simulink model "quadrotor_model"  (R2024b)
settings: Solver=VariableStepAuto  StartTime=0.0  StopTime=15  FixedStep=0.005  RelTol=1e-3
values from neighbouring files (symbols this model uses):
  Kd_phi = Cphi.Kd    [pidtune_baseline.m]
  Kd_psi = Cpsi.Kd    [pidtune_baseline.m]
  Kd_theta = Ctheta.Kd    [pidtune_baseline.m]
  Kd_z = Cz.Kd    [pidtune_baseline.m]
  Ki_phi = Cphi.Ki    [pidtune_baseline.m]
  Ki_psi = Cpsi.Ki    [pidtune_baseline.m]
  Ki_theta = Ctheta.Ki    [pidtune_baseline.m]
  Ki_z = Cz.Ki    [pidtune_baseline.m]
  Kp_phi = Cphi.Kp    [pidtune_baseline.m]
  Kp_psi = Cpsi.Kp    [pidtune_baseline.m]
  Kp_theta = Ctheta.Kp    [pidtune_baseline.m]
  Kp_z = Cz.Kp    [pidtune_baseline.m]
  l = 0.225    [motor_forward.m]
undefined symbols (not defined in the file or in its folder): altitude_d, altitude_i, b, g, I_xx, I_yy, I_zz, Im, k, m, pitch_d, pitch_i, roll_d, roll_i, yaw_d, yaw_i
libraries: slpidlib x4
settings Model: Creator=angel  LastModifiedBy=Yusuf
settings SolverCC: AlgebraicLoopSolver=TrustRegion
settings DataIOCC: ReturnWorkspaceOutputs=off
settings DebuggingCC: UnconnectedInputMsg=warning  UnconnectedOutputMsg=warning  UnconnectedLineMsg=warning  ArithmeticOperatorsInVariantConditions=warning
settings ModelReferenceCC: EnableRefExpFcnMdlSchedulingChecks=on
settings SFSimCC: SimUseLocalCustomCode=off  CustomCodeUndefinedFunction=UseInterfaceOnly
settings RTWCC: RTWUseLocalCustomCode=off  GPUComputeCapability=3.5
settings CodeAppCC: StateflowObjectComments=on

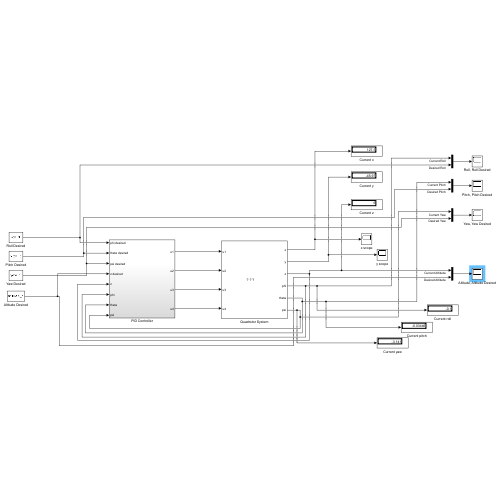
[thumbnail: Simulink's stored preview of the top-level diagram]
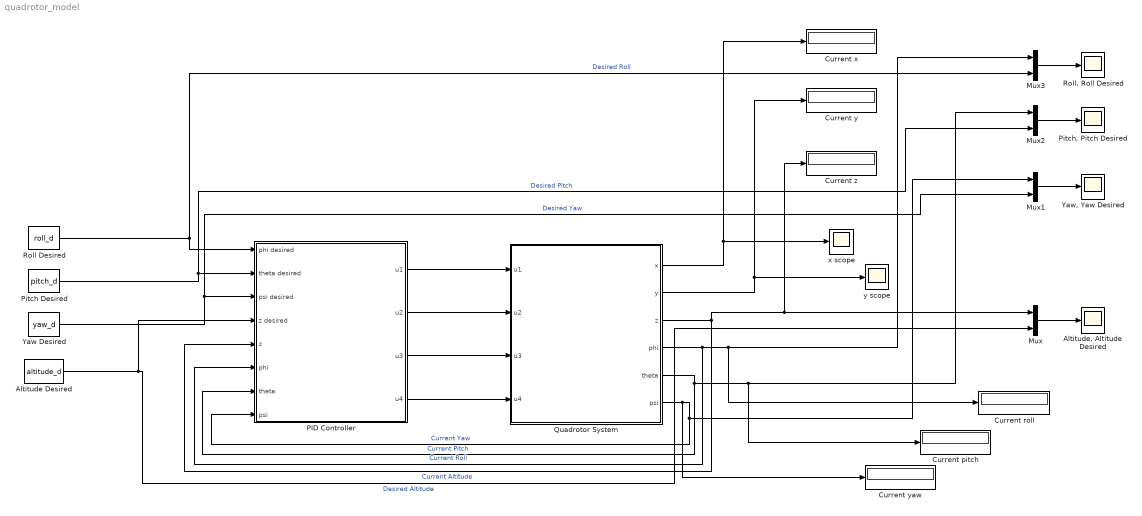
== system quadrotor_model ==
  Altitude Desired : Constant  Value=altitude_d
  "Altitude, Altitude Desired" : Scope
  Current pitch : Display
  Current roll : Display
  Current x : Display
  Current y : Display
  Current yaw : Display
  Current z : Display
  Mux{,1..3} (4 alike) : Mux  Inputs=2
  PID Controller : Subsystem
  Pitch Desired : Constant  Value=pitch_d
  "Pitch, Pitch Desired" : Scope
  Quadrotor System : Subsystem
      mask Display: image('C:\Users\angel\OneDrive - Universidad Politécnica de Yucatán\CIMAT\1st semester\Robotic Systems Modeling and Control\Project\Quadrotor\images\quadrotor.jpg');
  Roll Desired : Constant  Value=roll_d
  "Roll, Roll Desired" : Scope
  Yaw Desired : Constant  Value=yaw_d
  "Yaw, Yaw Desired" : Scope
  x scope : Scope
  y scope : Scope
  wires:
  Quadrotor System/1(x) -> x scope/1, Current x/1
  Quadrotor System/2(y) -> Current y/1, y scope/1
  Quadrotor System/3(z) -> Current z/1, Mux/1, PID Controller/5(z)  "Current Altitude"
  Quadrotor System/5(theta) -> Mux2/1, Current pitch/1, PID Controller/7(theta)  "Current Pitch"
  Quadrotor System/6(psi) -> Current yaw/1, Mux1/1, PID Controller/8(psi)  "Current Yaw"
  Mux/1 -> "Altitude, Altitude Desired"/1
  Roll Desired/1 -> Mux3/2, PID Controller/1(phi desired)  "Desired Roll"
  Pitch Desired/1 -> Mux2/2, PID Controller/2(theta desired)  "Desired Pitch"
  Yaw Desired/1 -> Mux1/2, PID Controller/3(psi desired)  "Desired Yaw"
  Quadrotor System/4(phi) -> PID Controller/6(phi), Current roll/1, Mux3/1  "Current Roll"
  Mux2/1 -> "Pitch, Pitch Desired"/1
  Mux1/1 -> "Yaw, Yaw Desired"/1
  Mux3/1 -> "Roll, Roll Desired"/1
  Altitude Desired/1 -> PID Controller/4(z desired), Mux/2  "Desired Altitude"
  PID Controller/1(u1) -> Quadrotor System/1(u1)
  PID Controller/2(u2) -> Quadrotor System/2(u2)
  PID Controller/3(u3) -> Quadrotor System/3(u3)
  PID Controller/4(u4) -> Quadrotor System/4(u4)

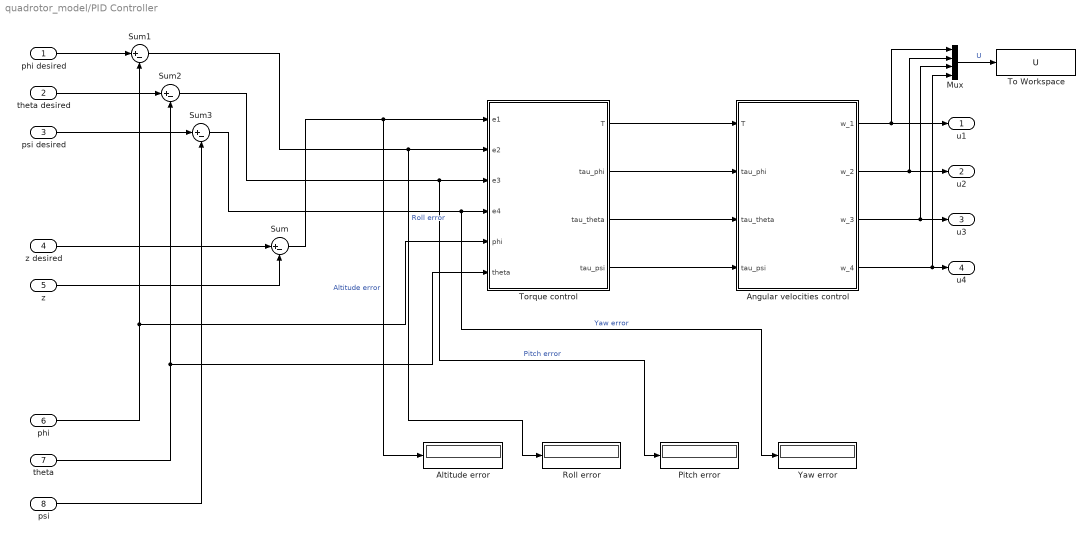
== system quadrotor_model/PID Controller ==
  phi desired : Inport
  theta desired : Inport  Port=2
  psi desired : Inport  Port=3
  z desired : Inport  Port=4
  z : Inport  Port=5
  phi : Inport  Port=6
  theta : Inport  Port=7
  psi : Inport  Port=8
  Altitude error : Display
  Angular velocities control : Subsystem
  Mux : Mux
  Pitch error : Display
  Roll error : Display
  Sum{,1..3} (4 alike) : Sum  Inputs=|+-
  To Workspace : ToWorkspace  VariableName=U  SaveFormat=Timeseries  SampleTime=-1
  Torque control : Subsystem
  Yaw error : Display
  u1 : Outport
  u2 : Outport  Port=2
  u3 : Outport  Port=3
  u4 : Outport  Port=4
  wires:
  z desired/1 -> Sum/1
  z/1 -> Sum/2
  Sum/1 -> Altitude error/1, Torque control/1(e1)  "Altitude error"
  phi desired/1 -> Sum1/1
  phi/1 -> Torque control/5("phi "), Sum1/2
  theta desired/1 -> Sum2/1
  theta/1 -> Sum2/2, Torque control/6("theta ")
  psi desired/1 -> Sum3/1
  psi/1 -> Sum3/2
  Sum1/1 -> Roll error/1, Torque control/2(e2)  "Roll error"
  Sum2/1 -> Pitch error/1, Torque control/3(e3)  "Pitch error"
  Sum3/1 -> Yaw error/1, Torque control/4(e4)  "Yaw error"
  Torque control/2(tau_phi) -> Angular velocities control/2(tau_phi)
  Torque control/1(T) -> Angular velocities control/1(T)
  Torque control/3(tau_theta) -> Angular velocities control/3(tau_theta)
  Torque control/4(tau_psi) -> Angular velocities control/4("tau_psi ")
  Angular velocities control/1(w_1) -> Mux/1, u1/1
  Angular velocities control/2(w_2) -> Mux/2, u2/1
  Angular velocities control/3(w_3) -> Mux/3, u3/1
  Angular velocities control/4("w_4 ") -> Mux/4, u4/1
  Mux/1 -> To Workspace/1  "U"

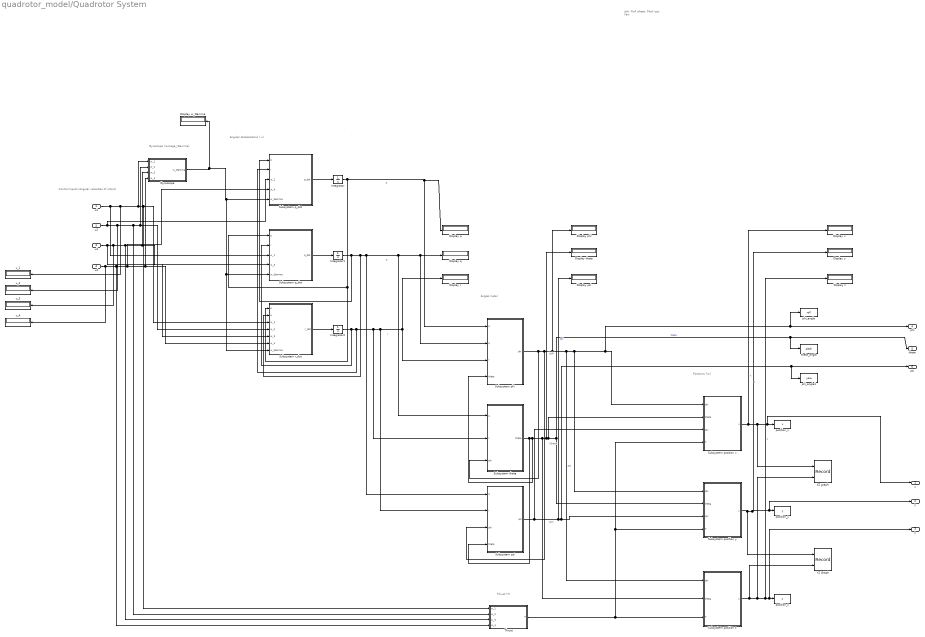
== system quadrotor_model/Quadrotor System ==
  note: Angular Accelerations (\nu)
  note: .
  note: \phi: Roll
      | \theta: Pitch
      | \psi: Yaw
  note: Control Inputs
      | (Angular velocities of rotors)
  note: Positions (\xi)
  note: Angles (\eta)
  note: Gyroscope (\omega_\Gamma)
  note: Thrust (T)
  note: p
  note: q
  note: r
  note: \phi
  note: \theta
  note: \psi
  u1 : Inport
  u2 : Inport  Port=2
  u3 : Inport  Port=3
  u4 : Inport  Port=4
  Display p : Display
  Display phi : Display
  Display psi : Display
  Display q : Display
  Display r : Display
  Display theta : Display
  Display w_Gamma : Display
  Display x : Display
  Display y : Display
  Display z : Display
  Gyroscope : MATLAB Function  TreatAsAtomicUnit=on
  Integrator : Integrator
  Integrator1 : Integrator
  Integrator2 : Integrator
  Subsystem p_dot : Subsystem
  Subsystem phi : Subsystem
  Subsystem position x : Subsystem
  Subsystem position y : Subsystem
  Subsystem position z : Subsystem
  Subsystem psi : Subsystem
  Subsystem q_dot : Subsystem
  Subsystem r_dot : Subsystem
  Subsystem theta : Subsystem
  Thrust : MATLAB Function  TreatAsAtomicUnit=on
  XZ graph : Record  FileSettingsInternal="{\"entries\":[{\"content\":{\"excelSettings\":{\"content\":{},\"type\":\"Streamout.ExcelSettings\"}},\"type\":\"Streamout.FileSettingStorage\",\"uuid\":\"\"}],\"packageUris\":[\"http:\\/\\/schema.mathworks.com\\/mf0\\/streamout_blocks\\/R2020a\"],\"version\":\"1.0\"}"  Layout=[1 1]  SignalsInternal="{\"entries\":[{\"content\":{\"signals\":[{\"content\":{\"blockPath\":[],\"dimensions\":[1],\"domain\":\"\",\"lineColor\":\"#a2142f\",\"plots\":[ 1 ],\"port\":1,\"sid\":[\"\"],\"signalID\":1,\"signalName\":\"x\"},\"type\":\"RecordBlkView.Signal\",\"uuid\":\"\"},{\"content\":{\"blockPath\":[],\"dimensions\":[1],\"domain\":\"\",\"lineColor\":\"#139fff\",\"plots\":[ 1 ],\"port\":2,\"sid\":[\"\"],\"signalID\":2,\"signalName\":\"z\"},\"type\":\"RecordBlkView.Signal\",\"uuid\":\"\"}]},\"type\":\"RecordBlkView.InputSignals\",\"uuid\":\"\"}],\"packageUris\":[\"http:\\/\\/schema.mathworks.com\\/mf0\\/streamout_blocks\\/R2020a\"],\"version\":\"1.0\"}"  VisualizationBindings="{\"xyplotplugin\":{\"info\":[{\"series\":[{\"bindingParametersList\":[{\"parameter\":\"X-Axis\",\"signalID\":1,\"signalName\":\"x\"},{\"parameter\":\"Y-Axis\",\"signalID\":2,\"signalName\":\"z\"}],\"seriesID\":0}],\"subplotID\":1}]}}"  CompatibilityTag=XY  st=-1
  YZ Graph : Record  FileSettingsInternal="{\"entries\":[{\"content\":{\"excelSettings\":{\"content\":{},\"type\":\"Streamout.ExcelSettings\"}},\"type\":\"Streamout.FileSettingStorage\",\"uuid\":\"\"}],\"packageUris\":[\"http:\\/\\/schema.mathworks.com\\/mf0\\/streamout_blocks\\/R2020a\"],\"version\":\"1.0\"}"  Layout=[1 1]  SignalsInternal="{\"entries\":[{\"content\":{\"signals\":[{\"content\":{\"blockPath\":[],\"dimensions\":[1],\"domain\":\"\",\"lineColor\":\"#a2142f\",\"plots\":[ 1 ],\"port\":1,\"sid\":[\"\"],\"signalID\":1,\"signalName\":\"y\"},\"type\":\"RecordBlkView.Signal\",\"uuid\":\"\"},{\"content\":{\"blockPath\":[],\"dimensions\":[1],\"domain\":\"\",\"lineColor\":\"#139fff\",\"plots\":[ 1 ],\"port\":2,\"sid\":[\"\"],\"signalID\":2,\"signalName\":\"z\"},\"type\":\"RecordBlkView.Signal\",\"uuid\":\"\"}]},\"type\":\"RecordBlkView.InputSignals\",\"uuid\":\"\"}],\"packageUris\":[\"http:\\/\\/schema.mathworks.com\\/mf0\\/streamout_blocks\\/R2020a\"],\"version\":\"1.0\"}"  VisualizationBindings="{\"xyplotplugin\":{\"info\":[{\"series\":[{\"bindingParametersList\":[{\"parameter\":\"X-Axis\",\"signalID\":1,\"signalName\":\"y\"},{\"parameter\":\"Y-Axis\",\"signalID\":2,\"signalName\":\"z\"}],\"seriesID\":0}],\"subplotID\":1}]}}"  CompatibilityTag=XY  st=-1
  phi_angle : ToWorkspace  VariableName=roll  SampleTime=-1
  phi_angle1 : ToWorkspace  VariableName=yaw  SampleTime=-1
  position_x : ToWorkspace  VariableName=x  SampleTime=-1
  position_y : ToWorkspace  VariableName=y  SampleTime=-1
  position_z : ToWorkspace  VariableName=z  SampleTime=-1
  theta_angle : ToWorkspace  VariableName=pitch  SampleTime=-1
  u_{1..4} (4 alike) : Display
  x : Outport
  y : Outport  Port=2
  z : Outport  Port=3
  phi : Outport  Port=4
  theta : Outport  Port=5
  psi : Outport  Port=6
  wires:
  u1/1 -> Subsystem q_dot/3(w_1), u_1/1, Gyroscope/1(w_1), Subsystem r_dot/3(w_1), Thrust/1(w_1)
  u2/1 -> Subsystem p_dot/3(w_2), u_2/1, Gyroscope/2(w_2), Subsystem r_dot/4(w_2), Thrust/2(w_2)
  u3/1 -> Subsystem q_dot/4(w_3), Gyroscope/3(w_3), Subsystem r_dot/5(w_3), Thrust/3(w_3), u_3/1
  u4/1 -> u_4/1, Gyroscope/4(w_4), Subsystem r_dot/6(w_4), Subsystem p_dot/4(w_4), Thrust/4(w_4)
  Thrust/1(T) -> Subsystem position y/4("T "), Subsystem position x/4(T), Subsystem position z/3(T)
  Subsystem phi/1("phi ") -> Subsystem theta/3("phi "), Subsystem psi/3(phi), Display phi/1, Subsystem position z/1("phi "), Subsystem position y/1("phi "), phi_angle/1, phi/1, Subsystem position x/1("phi ")  "phi"
  Subsystem psi/1(psi) -> Subsystem position x/3("psi "), Display psi/1, phi_angle1/1, psi/1, Subsystem position y/3("psi ")  "psi"
  Subsystem position x/1(x) -> Display x/1, x/1, position_x/1, XZ graph/1  "x"
  Subsystem position z/1(z) -> YZ Graph/2, XZ graph/2, z/1, position_z/1, Display z/1  "z"
  Subsystem position y/1("y ") -> y/1, position_y/1, Display y/1, YZ Graph/1  "y"
  Gyroscope/1(w_Gamma) -> Display w_Gamma/1, Subsystem r_dot/7(w_Gamma), Subsystem q_dot/5("w_Gamma "), Subsystem p_dot/5("w_Gamma ")
  Subsystem p_dot/1(p_dot) -> Integrator/1
  Subsystem q_dot/1(q_dot) -> Integrator1/1
  Subsystem r_dot/1(r_dot) -> Integrator2/1
  Integrator/1 -> Subsystem r_dot/1("p "), Subsystem q_dot/1("p "), Display p/1, Subsystem phi/1(p)
  Integrator2/1 -> Subsystem theta/2(r), Subsystem psi/2(r), Display r/1, Subsystem phi/3(r), Subsystem p_dot/2(r), Subsystem q_dot/2(r)
  Integrator1/1 -> Subsystem p_dot/1(q), Subsystem psi/1(q), Subsystem theta/1(q), Display q/1, Subsystem phi/2(q), Subsystem r_dot/2(q)
  Subsystem theta/1(theta) -> Subsystem psi/4(theta), Subsystem phi/4(theta), Subsystem position z/2("theta "), Display theta/1, Subsystem position x/2("theta "), theta_angle/1, theta/1, Subsystem position y/2("theta ")  "theta"

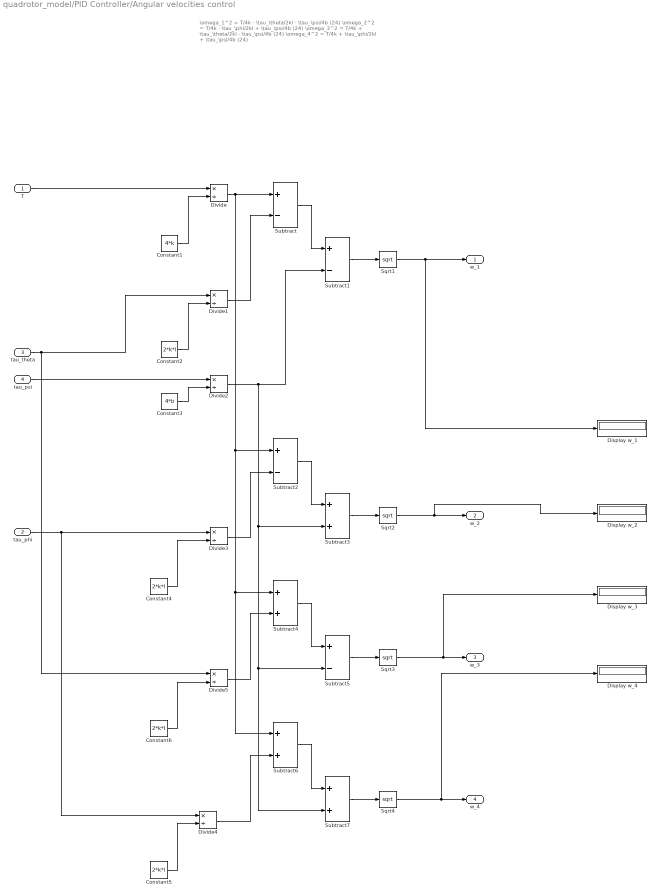
== system quadrotor_model/PID Controller/Angular velocities control ==
  note: \omega_1^2 = T/4k - \tau_\theta/2kl - \tau_\psi/4b   (24)
      |
      | \omega_2^2 = T/4k - \tau_\phi/2kl + \tau_\psi/4b   (24)
      |
      | \omega_3^2 = T/4k + \tau_\theta/2kl - \tau_\psi/4b   (24)
      |
      | \omega_4^2 = T/4k + \tau_\phi/2kl + \tau_\psi/4b   (24)
  T : Inport
  tau_phi : Inport  Port=2
  tau_theta : Inport  Port=3
  "tau_psi " : Inport  Port=4
  Constant1 : Constant  Value=4*k
  Constant{2,4..6} (4 alike) : Constant  Value=2*k*l
  Constant3 : Constant  Value=4*b
  Display w_{1..4} (4 alike) : Display
  Divide{,1..5} (6 alike) : Product  Inputs=*/
  Sqrt1 : Sqrt
  Sqrt2 : Sqrt  OutputSignalType=real
  Sqrt3 : Sqrt
  Sqrt4 : Sqrt
  Subtract{,1..2,5} (4 alike) : Sum  Inputs=+-
  Subtract{3..4,6..7} (4 alike) : Sum
  w_1 : Outport
  w_2 : Outport  Port=2
  w_3 : Outport  Port=3
  "w_4 " : Outport  Port=4
  wires:
  Constant1/1 -> Divide/2
  T/1 -> Divide/1
  Divide/1 -> Subtract4/1, Subtract6/1, Subtract2/1, Subtract/1
  Constant2/1 -> Divide1/2
  tau_theta/1 -> Divide5/1, Divide1/1
  Divide1/1 -> Subtract/2
  Subtract/1 -> Subtract1/1
  Constant3/1 -> Divide2/2
  Subtract1/1 -> Sqrt1/1
  Sqrt1/1 -> Display w_1/1, w_1/1
  Constant4/1 -> Divide3/2
  tau_phi/1 -> Divide4/1, Divide3/1
  Divide3/1 -> Subtract2/2
  Subtract2/1 -> Subtract3/1
  "tau_psi "/1 -> Divide2/1
  Divide2/1 -> Subtract7/2, Subtract5/2, Subtract3/2, Subtract1/2
  Sqrt2/1 -> Display w_2/1, w_2/1
  Subtract3/1 -> Sqrt2/1
  Constant6/1 -> Divide5/2
  Divide5/1 -> Subtract4/2
  Subtract5/1 -> Sqrt3/1
  Subtract4/1 -> Subtract5/1
  Sqrt3/1 -> Display w_3/1, w_3/1
  Subtract7/1 -> Sqrt4/1
  Constant5/1 -> Divide4/2
  Divide4/1 -> Subtract6/2
  Subtract6/1 -> Subtract7/1
  Sqrt4/1 -> Display w_4/1, "w_4 "/1

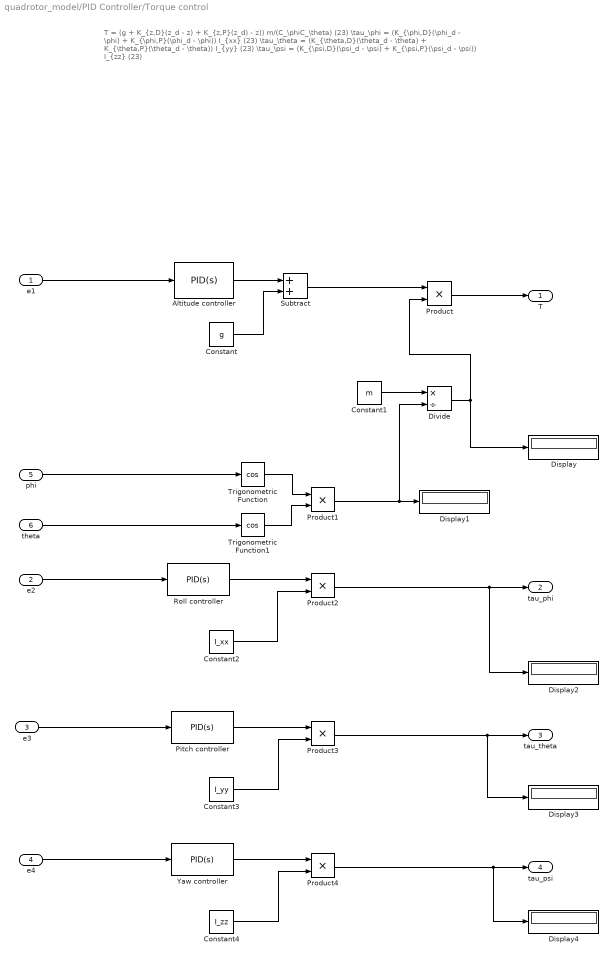
== system quadrotor_model/PID Controller/Torque control ==
  note: T = (g + K_{z,D}(z_d - z) + K_{z,P}(z_d) - z)) m/(C_\phiC_\theta)     (23)
      |
      | \tau_\phi = (K_{\phi,D}(\phi_d - \phi) + K_{\phi,P}(\phi_d - \phi)) I_{xx}                   (23)
      |
      | \tau_\theta = (K_{\theta,D}(\theta_d - \theta) + K_{\theta,P}(\theta_d - \theta)) I_{yy}                    (23)
      |
      | \tau_\psi = (K_{\psi,D}(\psi_d - \psi) + K_{\psi,P}(\psi_d - \psi)) I_{zz}                (23)
  e1 : Inport
  e2 : Inport  Port=2
  e3 : Inport  Port=3
  e4 : Inport  Port=4
  "phi " : Inport  Port=5
  "theta " : Inport  Port=6
  Altitude controller : slpidlib/PID Controller  Controller=PID  Form=Parallel  TimeDomain=Continuous-time  UseExternalTs=off  SampleTime=-1  IntegratorMethod=Forward Euler  FilterMethod=Forward Euler  ControllerParametersSource=internal  P=Kp_z  I=Ki_z  UseKiTs=off  D=Kd_z  UseExternalDerivativeSource=off  N=572.770791824146  UseFilter=on  TunerSelectOption=Transfer Function Based (PID Tuner App)  InitialConditionSource=internal  InitialConditionForIntegrator=0  InitialConditionForFilter=0  DifferentiatorICPrevScaledInput=0  ExternalReset=none  TrackingMode=off  Kt=1  LimitOutput=on  SatLimitsSource=internal  UpperSaturationLimit=5  LowerSaturationLimit=-5  LinearizeAsGain=on  AntiWindupMode=none  Kb=1  LimitIntegrator=off  UpperIntegratorSaturationLimit=inf  LowerIntegratorSaturationLimit=-inf  POutMin=[]  POutMax=[]  IOutMin=[]  IOutMax=[]  DOutMin=[]  DOutMax=[]  NOutMin=[]  NOutMax=[]  SumOutMin=[]  SumOutMax=[]  SaturationOutMin=[]  SaturationOutMax=[]  PParamMin=[]  PParamMax=[]  IParamMin=[]  IParamMax=[]  DParamMin=[]  DParamMax=[]  NParamMin=[]  NParamMax=[]  KbParamMin=[]  KbParamMax=[]  KtParamMin=[]  KtParamMax=[]  KbOutMin=[]  KbOutMax=[]  KtOutMin=[]  KtOutMax=[]  IntegratorOutMin=[]  IntegratorOutMax=[]  FilterOutMin=[]  FilterOutMax=[]  SumI1OutMin=[]  SumI1OutMax=[]  SumI2OutMin=[]  SumI2OutMax=[]  SumI3OutMin=[]  SumI3OutMax=[]  SumI4OutMin=[]  SumI4OutMax=[]  SumDOutMin=[]  SumDOutMax=[]  DifferentiatorOutMin=[]  DifferentiatorOutMax=[]  FilterDiffOutCoefMin=[]  FilterDiffOutCoefMax=[]  ReciprocalOutMin=[]  ReciprocalOutMax=[]  SumDenOutMin=[]  SumDenOutMax=[]  SumNumOutMin=[]  SumNumOutMax=[]  DivideOutMin=[]  DivideOutMax=[]  UdiffTsProdOutMin=[]  UdiffTsProdOutMax=[]  NTsProdOutMin=[]  NTsProdOutMax=[]  UintegralTsProdOutMin=[]  UintegralTsProdOutMax=[]  UngainTsProdOutMin=[]  UngainTsProdOutMax=[]  ClampingZeroOutDataTypeStr=Inherit: Inherit via back propagation  ClampingZeroOutMin=[]  ClampingZeroOutMax=[]  FilterDenConstantOutDataTypeStr=Inherit: Inherit via back propagation  FilterDenConstantOutMin=[]  FilterDenConstantOutMax=[]  PCopyOutDataTypeStr=Inherit: Inherit via back propagation  PCopyOutMin=[]  PCopyOutMax=[]  NCopyOutDataTypeStr=Inherit: Inherit via back propagation  NCopyOutMin=[]  NCopyOutMax=[]  IntegratorContinuousStateAttributes=''  IntegratorStateMustResolveToSignalObject=off  IntegratorRTWStateStorageClass=Auto  FilterContinuousStateAttributes=''  FilterStateMustResolveToSignalObject=off  FilterRTWStateStorageClass=Auto  ParallelPVariant=InternalParameters  IdealPVariant=Disabled  IVariant=InternalParameters  DVariant=InternalParameters  IntegratorVariant=Continuous  SatVariant=Enabled  AWVariant=Passthrough  PCopyVariant=Disabled  TRVariant=Disabled  FdbkBlocksVariant=Forward  IdealPFdbkVariant=Disabled  SatFdbkVariant=Disabled  DerivativeFilterVariant=ContFilter  NVariant=InternalParameters  NCopyVariant=Disabled  FilterICVariant=InternalICsFilter  IntegratorICVariant=InternalICs  ExternalResetVariant=Disabled  TRSumVariant=Passthrough  SumFdbkVariant=Disabled  SumVariant=Sum_PID  TsampFilterVariant=InternalTs  TsampNgainVariant=Passthrough  TsampIntegralVariant=Disabled_SignalSpec  ExternalSaturationOutDataTypeStr=Inherit: Same as second input  DerivativeSourceVariant=ErrorSignal  PreIntVariant=InternalPreInt
  Constant : Constant  Value=g
  Constant1 : Constant  Value=m
  Constant2 : Constant  Value=I_xx
  Constant3 : Constant  Value=I_yy
  Constant4 : Constant  Value=I_zz
  Display{,1..4} (5 alike) : Display
  Divide : Product  Inputs=*/
  Pitch controller : slpidlib/PID Controller  Controller=PID  Form=Parallel  TimeDomain=Continuous-time  UseExternalTs=off  SampleTime=-1  IntegratorMethod=Forward Euler  FilterMethod=Forward Euler  ControllerParametersSource=internal  P=Kp_theta  I=Ki_theta  UseKiTs=off  D=Kd_theta  UseExternalDerivativeSource=off  N=1414.64809761679  UseFilter=on  TunerSelectOption=Transfer Function Based (PID Tuner App)  InitialConditionSource=internal  InitialConditionForIntegrator=0  InitialConditionForFilter=0  DifferentiatorICPrevScaledInput=0  ExternalReset=none  TrackingMode=off  Kt=1  LimitOutput=on  SatLimitsSource=internal  UpperSaturationLimit=0.9  LowerSaturationLimit=-0.9  LinearizeAsGain=on  AntiWindupMode=none  Kb=1  LimitIntegrator=off  UpperIntegratorSaturationLimit=inf  LowerIntegratorSaturationLimit=-inf  POutMin=[]  POutMax=[]  IOutMin=[]  IOutMax=[]  DOutMin=[]  DOutMax=[]  NOutMin=[]  NOutMax=[]  SumOutMin=[]  SumOutMax=[]  SaturationOutMin=[]  SaturationOutMax=[]  PParamMin=[]  PParamMax=[]  IParamMin=[]  IParamMax=[]  DParamMin=[]  DParamMax=[]  NParamMin=[]  NParamMax=[]  KbParamMin=[]  KbParamMax=[]  KtParamMin=[]  KtParamMax=[]  KbOutMin=[]  KbOutMax=[]  KtOutMin=[]  KtOutMax=[]  IntegratorOutMin=[]  IntegratorOutMax=[]  FilterOutMin=[]  FilterOutMax=[]  SumI1OutMin=[]  SumI1OutMax=[]  SumI2OutMin=[]  SumI2OutMax=[]  SumI3OutMin=[]  SumI3OutMax=[]  SumI4OutMin=[]  SumI4OutMax=[]  SumDOutMin=[]  SumDOutMax=[]  DifferentiatorOutMin=[]  DifferentiatorOutMax=[]  FilterDiffOutCoefMin=[]  FilterDiffOutCoefMax=[]  ReciprocalOutMin=[]  ReciprocalOutMax=[]  SumDenOutMin=[]  SumDenOutMax=[]  SumNumOutMin=[]  SumNumOutMax=[]  DivideOutMin=[]  DivideOutMax=[]  UdiffTsProdOutMin=[]  UdiffTsProdOutMax=[]  NTsProdOutMin=[]  NTsProdOutMax=[]  UintegralTsProdOutMin=[]  UintegralTsProdOutMax=[]  UngainTsProdOutMin=[]  UngainTsProdOutMax=[]  ClampingZeroOutDataTypeStr=Inherit: Inherit via back propagation  ClampingZeroOutMin=[]  ClampingZeroOutMax=[]  FilterDenConstantOutDataTypeStr=Inherit: Inherit via back propagation  FilterDenConstantOutMin=[]  FilterDenConstantOutMax=[]  PCopyOutDataTypeStr=Inherit: Inherit via back propagation  PCopyOutMin=[]  PCopyOutMax=[]  NCopyOutDataTypeStr=Inherit: Inherit via back propagation  NCopyOutMin=[]  NCopyOutMax=[]  IntegratorContinuousStateAttributes=''  IntegratorStateMustResolveToSignalObject=off  IntegratorRTWStateStorageClass=Auto  FilterContinuousStateAttributes=''  FilterStateMustResolveToSignalObject=off  FilterRTWStateStorageClass=Auto  ParallelPVariant=InternalParameters  IdealPVariant=Disabled  IVariant=InternalParameters  DVariant=InternalParameters  IntegratorVariant=Continuous  SatVariant=Enabled  AWVariant=Passthrough  PCopyVariant=Disabled  TRVariant=Disabled  FdbkBlocksVariant=Forward  IdealPFdbkVariant=Disabled  SatFdbkVariant=Disabled  DerivativeFilterVariant=ContFilter  NVariant=InternalParameters  NCopyVariant=Disabled  FilterICVariant=InternalICsFilter  IntegratorICVariant=InternalICs  ExternalResetVariant=Disabled  TRSumVariant=Passthrough  SumFdbkVariant=Disabled  SumVariant=Sum_PID  TsampFilterVariant=InternalTs  TsampNgainVariant=Passthrough  TsampIntegralVariant=Disabled_SignalSpec  ExternalSaturationOutDataTypeStr=Inherit: Same as second input  DerivativeSourceVariant=ErrorSignal  PreIntVariant=InternalPreInt
  Product{,1..4} (5 alike) : Product
  Roll controller : slpidlib/PID Controller  Controller=PID  Form=Parallel  TimeDomain=Continuous-time  UseExternalTs=off  SampleTime=-1  IntegratorMethod=Forward Euler  FilterMethod=Forward Euler  ControllerParametersSource=internal  P=Kp_phi  I=Ki_phi  UseKiTs=off  D=Kd_phi  UseExternalDerivativeSource=off  N=1414.64809761679  UseFilter=on  TunerSelectOption=Transfer Function Based (PID Tuner App)  InitialConditionSource=internal  InitialConditionForIntegrator=0  InitialConditionForFilter=0  DifferentiatorICPrevScaledInput=0  ExternalReset=none  TrackingMode=off  Kt=1  LimitOutput=on  SatLimitsSource=internal  UpperSaturationLimit=0.9  LowerSaturationLimit=-0.9  LinearizeAsGain=on  AntiWindupMode=none  Kb=1  LimitIntegrator=off  UpperIntegratorSaturationLimit=inf  LowerIntegratorSaturationLimit=-inf  POutMin=[]  POutMax=[]  IOutMin=[]  IOutMax=[]  DOutMin=[]  DOutMax=[]  NOutMin=[]  NOutMax=[]  SumOutMin=[]  SumOutMax=[]  SaturationOutMin=[]  SaturationOutMax=[]  PParamMin=[]  PParamMax=[]  IParamMin=[]  IParamMax=[]  DParamMin=[]  DParamMax=[]  NParamMin=[]  NParamMax=[]  KbParamMin=[]  KbParamMax=[]  KtParamMin=[]  KtParamMax=[]  KbOutMin=[]  KbOutMax=[]  KtOutMin=[]  KtOutMax=[]  IntegratorOutMin=[]  IntegratorOutMax=[]  FilterOutMin=[]  FilterOutMax=[]  SumI1OutMin=[]  SumI1OutMax=[]  SumI2OutMin=[]  SumI2OutMax=[]  SumI3OutMin=[]  SumI3OutMax=[]  SumI4OutMin=[]  SumI4OutMax=[]  SumDOutMin=[]  SumDOutMax=[]  DifferentiatorOutMin=[]  DifferentiatorOutMax=[]  FilterDiffOutCoefMin=[]  FilterDiffOutCoefMax=[]  ReciprocalOutMin=[]  ReciprocalOutMax=[]  SumDenOutMin=[]  SumDenOutMax=[]  SumNumOutMin=[]  SumNumOutMax=[]  DivideOutMin=[]  DivideOutMax=[]  UdiffTsProdOutMin=[]  UdiffTsProdOutMax=[]  NTsProdOutMin=[]  NTsProdOutMax=[]  UintegralTsProdOutMin=[]  UintegralTsProdOutMax=[]  UngainTsProdOutMin=[]  UngainTsProdOutMax=[]  ClampingZeroOutDataTypeStr=Inherit: Inherit via back propagation  ClampingZeroOutMin=[]  ClampingZeroOutMax=[]  FilterDenConstantOutDataTypeStr=Inherit: Inherit via back propagation  FilterDenConstantOutMin=[]  FilterDenConstantOutMax=[]  PCopyOutDataTypeStr=Inherit: Inherit via back propagation  PCopyOutMin=[]  PCopyOutMax=[]  NCopyOutDataTypeStr=Inherit: Inherit via back propagation  NCopyOutMin=[]  NCopyOutMax=[]  IntegratorContinuousStateAttributes=''  IntegratorStateMustResolveToSignalObject=off  IntegratorRTWStateStorageClass=Auto  FilterContinuousStateAttributes=''  FilterStateMustResolveToSignalObject=off  FilterRTWStateStorageClass=Auto  ParallelPVariant=InternalParameters  IdealPVariant=Disabled  IVariant=InternalParameters  DVariant=InternalParameters  IntegratorVariant=Continuous  SatVariant=Enabled  AWVariant=Passthrough  PCopyVariant=Disabled  TRVariant=Disabled  FdbkBlocksVariant=Forward  IdealPFdbkVariant=Disabled  SatFdbkVariant=Disabled  DerivativeFilterVariant=ContFilter  NVariant=InternalParameters  NCopyVariant=Disabled  FilterICVariant=InternalICsFilter  IntegratorICVariant=InternalICs  ExternalResetVariant=Disabled  TRSumVariant=Passthrough  SumFdbkVariant=Disabled  SumVariant=Sum_PID  TsampFilterVariant=InternalTs  TsampNgainVariant=Passthrough  TsampIntegralVariant=Disabled_SignalSpec  ExternalSaturationOutDataTypeStr=Inherit: Same as second input  DerivativeSourceVariant=ErrorSignal  PreIntVariant=InternalPreInt
  Subtract : Sum
  Trigonometric Function : Trigonometry  Operator=cos
  Trigonometric Function1 : Trigonometry  Operator=cos
  Yaw controller : slpidlib/PID Controller  Controller=PID  Form=Parallel  TimeDomain=Continuous-time  UseExternalTs=off  SampleTime=-1  IntegratorMethod=Forward Euler  FilterMethod=Forward Euler  ControllerParametersSource=internal  P=Kp_psi  I=Ki_psi  UseKiTs=off  D=Kd_psi  UseExternalDerivativeSource=off  N=95.667343116538  UseFilter=on  TunerSelectOption=Transfer Function Based (PID Tuner App)  InitialConditionSource=internal  InitialConditionForIntegrator=0  InitialConditionForFilter=0  DifferentiatorICPrevScaledInput=0  ExternalReset=none  TrackingMode=off  Kt=1  LimitOutput=on  SatLimitsSource=internal  UpperSaturationLimit=5  LowerSaturationLimit=-5  LinearizeAsGain=on  AntiWindupMode=none  Kb=1  LimitIntegrator=off  UpperIntegratorSaturationLimit=inf  LowerIntegratorSaturationLimit=-inf  POutMin=[]  POutMax=[]  IOutMin=[]  IOutMax=[]  DOutMin=[]  DOutMax=[]  NOutMin=[]  NOutMax=[]  SumOutMin=[]  SumOutMax=[]  SaturationOutMin=[]  SaturationOutMax=[]  PParamMin=[]  PParamMax=[]  IParamMin=[]  IParamMax=[]  DParamMin=[]  DParamMax=[]  NParamMin=[]  NParamMax=[]  KbParamMin=[]  KbParamMax=[]  KtParamMin=[]  KtParamMax=[]  KbOutMin=[]  KbOutMax=[]  KtOutMin=[]  KtOutMax=[]  IntegratorOutMin=[]  IntegratorOutMax=[]  FilterOutMin=[]  FilterOutMax=[]  SumI1OutMin=[]  SumI1OutMax=[]  SumI2OutMin=[]  SumI2OutMax=[]  SumI3OutMin=[]  SumI3OutMax=[]  SumI4OutMin=[]  SumI4OutMax=[]  SumDOutMin=[]  SumDOutMax=[]  DifferentiatorOutMin=[]  DifferentiatorOutMax=[]  FilterDiffOutCoefMin=[]  FilterDiffOutCoefMax=[]  ReciprocalOutMin=[]  ReciprocalOutMax=[]  SumDenOutMin=[]  SumDenOutMax=[]  SumNumOutMin=[]  SumNumOutMax=[]  DivideOutMin=[]  DivideOutMax=[]  UdiffTsProdOutMin=[]  UdiffTsProdOutMax=[]  NTsProdOutMin=[]  NTsProdOutMax=[]  UintegralTsProdOutMin=[]  UintegralTsProdOutMax=[]  UngainTsProdOutMin=[]  UngainTsProdOutMax=[]  ClampingZeroOutDataTypeStr=Inherit: Inherit via back propagation  ClampingZeroOutMin=[]  ClampingZeroOutMax=[]  FilterDenConstantOutDataTypeStr=Inherit: Inherit via back propagation  FilterDenConstantOutMin=[]  FilterDenConstantOutMax=[]  PCopyOutDataTypeStr=Inherit: Inherit via back propagation  PCopyOutMin=[]  PCopyOutMax=[]  NCopyOutDataTypeStr=Inherit: Inherit via back propagation  NCopyOutMin=[]  NCopyOutMax=[]  IntegratorContinuousStateAttributes=''  IntegratorStateMustResolveToSignalObject=off  IntegratorRTWStateStorageClass=Auto  FilterContinuousStateAttributes=''  FilterStateMustResolveToSignalObject=off  FilterRTWStateStorageClass=Auto  ParallelPVariant=InternalParameters  IdealPVariant=Disabled  IVariant=InternalParameters  DVariant=InternalParameters  IntegratorVariant=Continuous  SatVariant=Enabled  AWVariant=Passthrough  PCopyVariant=Disabled  TRVariant=Disabled  FdbkBlocksVariant=Forward  IdealPFdbkVariant=Disabled  SatFdbkVariant=Disabled  DerivativeFilterVariant=ContFilter  NVariant=InternalParameters  NCopyVariant=Disabled  FilterICVariant=InternalICsFilter  IntegratorICVariant=InternalICs  ExternalResetVariant=Disabled  TRSumVariant=Passthrough  SumFdbkVariant=Disabled  SumVariant=Sum_PID  TsampFilterVariant=InternalTs  TsampNgainVariant=Passthrough  TsampIntegralVariant=Disabled_SignalSpec  ExternalSaturationOutDataTypeStr=Inherit: Same as second input  DerivativeSourceVariant=ErrorSignal  PreIntVariant=InternalPreInt
  T : Outport
  tau_phi : Outport  Port=2
  tau_theta : Outport  Port=3
  tau_psi : Outport  Port=4
  wires:
  Constant/1 -> Subtract/2
  e1/1 -> Altitude controller/1
  Altitude controller/1 -> Subtract/1
  Subtract/1 -> Product/1
  Constant1/1 -> Divide/1
  Divide/1 -> Product/2, Display/1
  "phi "/1 -> Trigonometric Function/1
  "theta "/1 -> Trigonometric Function1/1
  Trigonometric Function/1 -> Product1/1
  Trigonometric Function1/1 -> Product1/2
  Product1/1 -> Display1/1, Divide/2
  Product/1 -> T/1
  e2/1 -> Roll controller/1
  Roll controller/1 -> Product2/1
  Constant2/1 -> Product2/2
  Product2/1 -> Display2/1, tau_phi/1
  Constant3/1 -> Product3/2
  Pitch controller/1 -> Product3/1
  Constant4/1 -> Product4/2
  Yaw controller/1 -> Product4/1
  e4/1 -> Yaw controller/1
  e3/1 -> Pitch controller/1
  Product3/1 -> Display3/1, tau_theta/1
  Product4/1 -> Display4/1, tau_psi/1

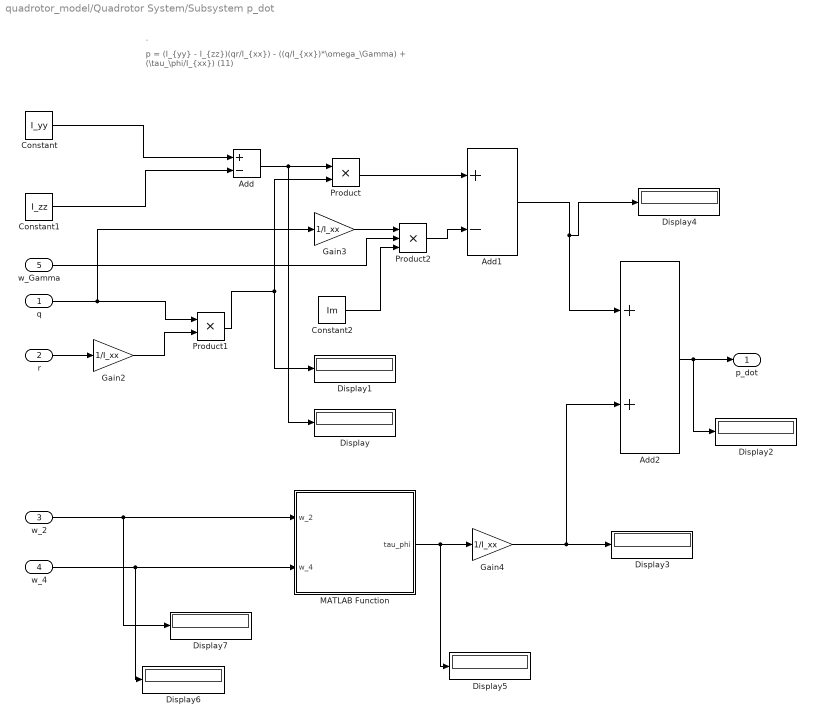
== system quadrotor_model/Quadrotor System/Subsystem p_dot ==
  note: p = (I_{yy} - I_{zz})(qr/I_{xx}) - ((q/I_{xx})*\omega_\Gamma) + (\tau_\phi/I_{xx}) (11)
  note: .
  q : Inport
  r : Inport  Port=2
  w_2 : Inport  Port=3
  w_4 : Inport  Port=4
  "w_Gamma " : Inport  Port=5
  Add : Sum  Inputs=+-
  Add1 : Sum  Inputs=+-
  Add2 : Sum
  Constant : Constant  Value=I_yy
  Constant1 : Constant  Value=I_zz
  Constant2 : Constant  Value=Im
  Display{,1..7} (8 alike) : Display
  Gain2 : Gain  Gain=1/I_xx
  Gain3 : Gain  Gain=1/I_xx
  Gain4 : Gain  Gain=1/I_xx
  MATLAB Function : MATLAB Function  TreatAsAtomicUnit=on
  Product : Product
  Product1 : Product
  Product2 : Product  Inputs=3
  p_dot : Outport
  wires:
  Constant/1 -> Add/1
  Constant1/1 -> Add/2
  Add/1 -> Display/1, Product/1
  Product/1 -> Add1/1
  Product2/1 -> Add1/2
  Add2/1 -> p_dot/1, Display2/1
  r/1 -> Gain2/1
  Gain2/1 -> Product1/2
  q/1 -> Gain3/1, Product1/1
  Gain3/1 -> Product2/1
  Product1/1 -> Display1/1, Product/2
  MATLAB Function/1(tau_phi) -> Display5/1, Gain4/1
  w_2/1 -> MATLAB Function/1(w_2), Display7/1
  w_4/1 -> Display6/1, MATLAB Function/2(w_4)
  "w_Gamma "/1 -> Product2/2
  Gain4/1 -> Display3/1, Add2/2
  Add1/1 -> Display4/1, Add2/1
  Constant2/1 -> Product2/3

== system quadrotor_model/Quadrotor System/Subsystem phi ==
  note: \phi
  note: \phi
  note: .
  note: \phi = p + q(S_\phiT_\theta) + r(C_\phiT_\theta) (4)
  note: .
  p : Inport
  q : Inport  Port=2
  r : Inport  Port=3
  theta : Inport  Port=4
  Display1 : Display
  Display10 : Display
  Display9 : Display
  Integrator6 : Integrator  InitialConditionSource=external  InitialCondition=-0.1
  Product5 : Product  Inputs=3
  Product6 : Product  Inputs=3
  Roll Initial : Constant  Value=roll_i
  Z''3 : Sum  Inputs=+++
  "cos " : Trigonometry  Operator=cos
  cos 1 : Trigonometry
  tan 1 : Trigonometry  Operator=tan
  tan 5 : Trigonometry  Operator=tan
  "phi " : Outport
  wires:
  "cos "/1 -> Product5/1
  Product5/1 -> Display10/1, Z''3/1
  theta/1 -> tan 5/1, tan 1/1
  Integrator6/1 -> "cos "/1, Display1/1, cos 1/1, "phi "/1
  tan 5/1 -> Product5/3
  Z''3/1 -> Integrator6/1
  q/1 -> Product6/2
  Product6/1 -> Display9/1, Z''3/3
  p/1 -> Z''3/2
  cos 1/1 -> Product6/1
  tan 1/1 -> Product6/3
  r/1 -> Product5/2
  Roll Initial/1 -> Integrator6/2

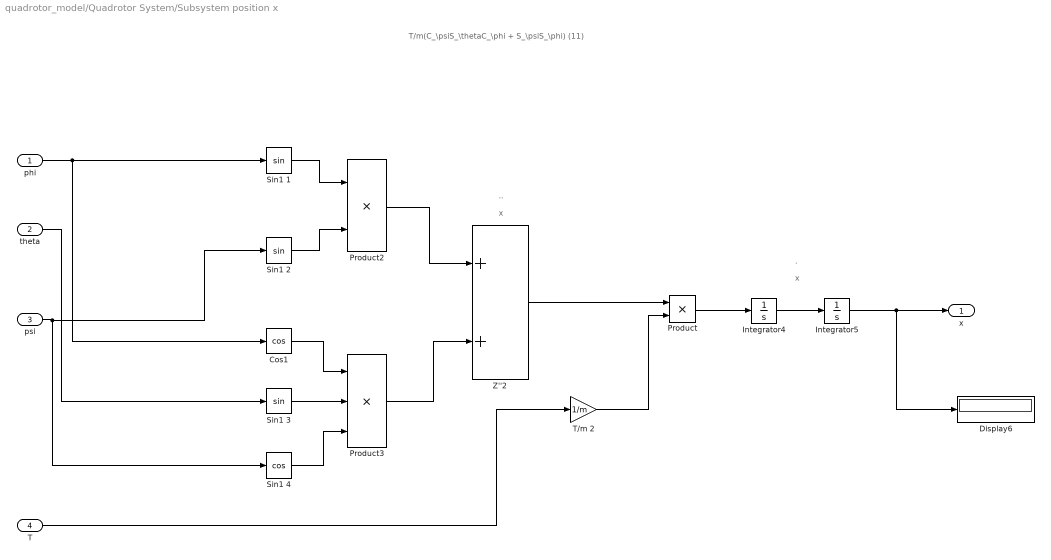
== system quadrotor_model/Quadrotor System/Subsystem position x ==
  note: ..
  note: x
  note: .
  note: x
  note: T/m(C_\psiS_\thetaC_\phi + S_\psiS_\phi) (11)
  "phi " : Inport
  "theta " : Inport  Port=2
  "psi " : Inport  Port=3
  T : Inport  Port=4
  Cos1 : Trigonometry  Operator=cos
  Display6 : Display
  Integrator4 : Integrator
  Integrator5 : Integrator
  Product : Product
  Product2 : Product
  Product3 : Product  Inputs=3
  Sin1 1 : Trigonometry
  Sin1 2 : Trigonometry
  Sin1 3 : Trigonometry
  Sin1 4 : Trigonometry  Operator=cos
  T/m 2 : Gain  Gain=1/m
  Z''2 : Sum
  x : Outport
  wires:
  "phi "/1 -> Cos1/1, Sin1 1/1
  "psi "/1 -> Sin1 2/1, Sin1 4/1
  Integrator4/1 -> Integrator5/1
  Product2/1 -> Z''2/1
  Product3/1 -> Z''2/2
  "theta "/1 -> Sin1 3/1
  Sin1 1/1 -> Product2/1
  Sin1 3/1 -> Product3/2
  Sin1 2/1 -> Product2/2
  Sin1 4/1 -> Product3/3
  Cos1/1 -> Product3/1
  Integrator5/1 -> x/1, Display6/1
  T/m 2/1 -> Product/2
  T/1 -> T/m 2/1
  Z''2/1 -> Product/1
  Product/1 -> Integrator4/1

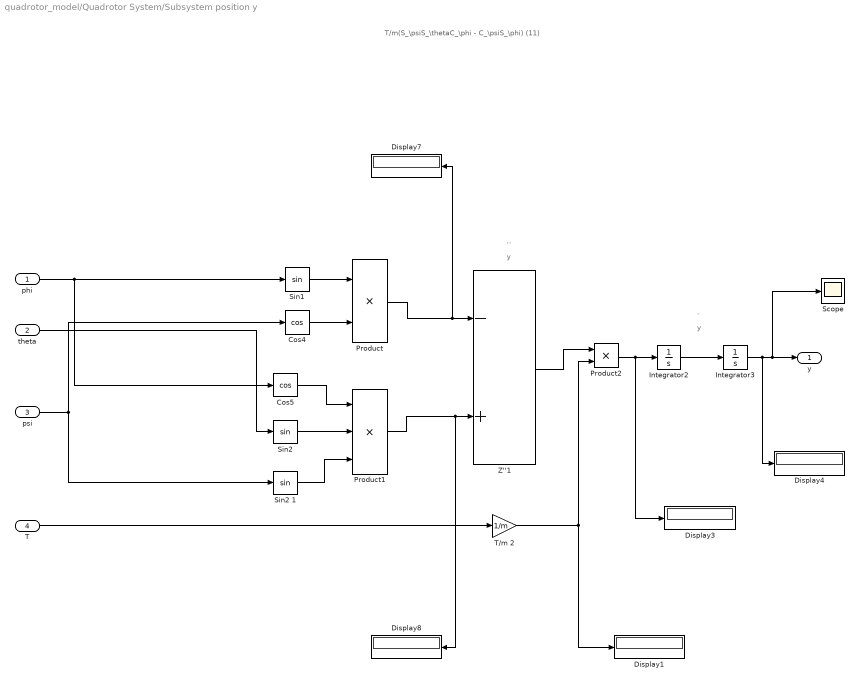
== system quadrotor_model/Quadrotor System/Subsystem position y ==
  note: T/m(S_\psiS_\thetaC_\phi - C_\psiS_\phi) (11)
  note: ..
  note: y
  note: y
  note: .
  "phi " : Inport
  "theta " : Inport  Port=2
  "psi " : Inport  Port=3
  "T " : Inport  Port=4
  Cos4 : Trigonometry  Operator=cos
  Cos5 : Trigonometry  Operator=cos
  Display{1,3..4,7..8} (5 alike) : Display
  Integrator2 : Integrator
  Integrator3 : Integrator
  Product : Product
  Product1 : Product  Inputs=3
  Product2 : Product
  Scope : Scope
  "Sin1 " : Trigonometry
  "Sin2 " : Trigonometry
  Sin2 1 : Trigonometry
  T/m 2 : Gain  Gain=1/m
  Z''1 : Sum  Inputs=-+
  "y " : Outport
  wires:
  Integrator2/1 -> Integrator3/1
  "theta "/1 -> "Sin2 "/1
  Integrator3/1 -> "y "/1, Scope/1, Display4/1
  "phi "/1 -> "Sin1 "/1, Cos5/1
  Product/1 -> Display7/1, Z''1/1
  Cos4/1 -> Product/2
  "psi "/1 -> Cos4/1, Sin2 1/1
  Sin2 1/1 -> Product1/3
  Product1/1 -> Display8/1, Z''1/2
  Cos5/1 -> Product1/1
  "Sin2 "/1 -> Product1/2
  "Sin1 "/1 -> Product/1
  "T "/1 -> T/m 2/1
  Z''1/1 -> Product2/1
  T/m 2/1 -> Display1/1, Product2/2
  Product2/1 -> Display3/1, Integrator2/1

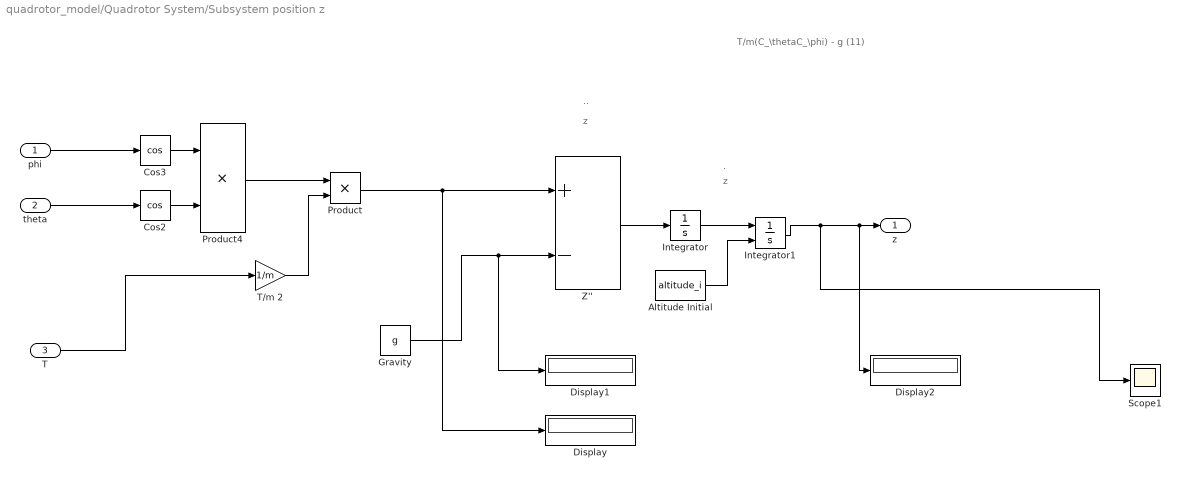
== system quadrotor_model/Quadrotor System/Subsystem position z ==
  note: z
  note: ..
  note: .
  note: z
  note: T/m(C_\thetaC_\phi) - g (11)
  "phi " : Inport
  "theta " : Inport  Port=2
  T : Inport  Port=3
  Altitude Initial : Constant  Value=altitude_i
  Cos2 : Trigonometry  Operator=cos
  Cos3 : Trigonometry  Operator=cos
  Display : Display
  Display1 : Display
  Display2 : Display
  Gravity : Constant  Value=g
  Integrator : Integrator
  Integrator1 : Integrator  InitialConditionSource=external
  Product : Product
  Product4 : Product
  Scope1 : Scope
  T/m 2 : Gain  Gain=1/m
  Z'' : Sum  Inputs=+-
  z : Outport
  wires:
  "phi "/1 -> Cos3/1
  Gravity/1 -> Display1/1, Z''/2
  Z''/1 -> Integrator/1
  Integrator1/1 -> z/1, Display2/1, Scope1/1
  "theta "/1 -> Cos2/1
  Integrator/1 -> Integrator1/1
  Cos2/1 -> Product4/2
  Cos3/1 -> Product4/1
  T/1 -> T/m 2/1
  Product4/1 -> Product/1
  Product/1 -> Display/1, Z''/1
  T/m 2/1 -> Product/2
  Altitude Initial/1 -> Integrator1/2

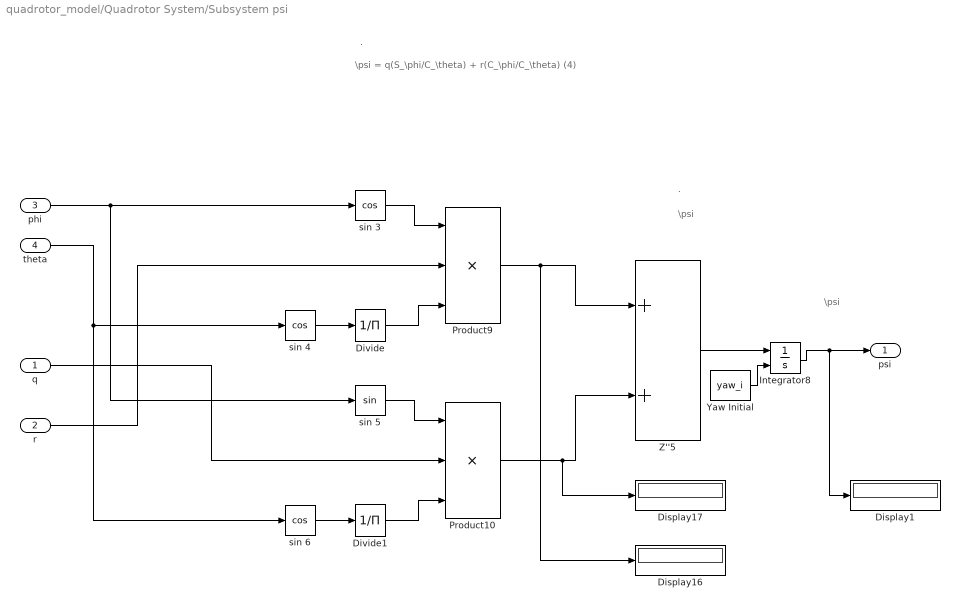
== system quadrotor_model/Quadrotor System/Subsystem psi ==
  note: .
  note: \psi
  note: \psi
  note: \psi = q(S_\phi/C_\theta) + r(C_\phi/C_\theta) (4)
  note: .
  q : Inport
  r : Inport  Port=2
  phi : Inport  Port=3
  theta : Inport  Port=4
  Display1 : Display
  Display16 : Display
  Display17 : Display
  Divide : Product  Inputs=/
  Divide1 : Product  Inputs=/
  Integrator8 : Integrator  InitialConditionSource=external  InitialCondition=-pi
  Product10 : Product  Inputs=3
  Product9 : Product  Inputs=3
  Yaw Initial : Constant  Value=yaw_i
  Z''5 : Sum
  sin 3 : Trigonometry  Operator=cos
  sin 4 : Trigonometry  Operator=cos
  sin 5 : Trigonometry
  sin 6 : Trigonometry  Operator=cos
  psi : Outport
  wires:
  sin 3/1 -> Product9/1
  Divide1/1 -> Product10/3
  sin 5/1 -> Product10/1
  sin 4/1 -> Divide/1
  Divide/1 -> Product9/3
  sin 6/1 -> Divide1/1
  Product9/1 -> Display16/1, Z''5/1
  theta/1 -> sin 6/1, sin 4/1
  phi/1 -> sin 5/1, sin 3/1
  q/1 -> Product10/2
  r/1 -> Product9/2
  Z''5/1 -> Integrator8/1
  Product10/1 -> Display17/1, Z''5/2
  Integrator8/1 -> Display1/1, psi/1
  Yaw Initial/1 -> Integrator8/2

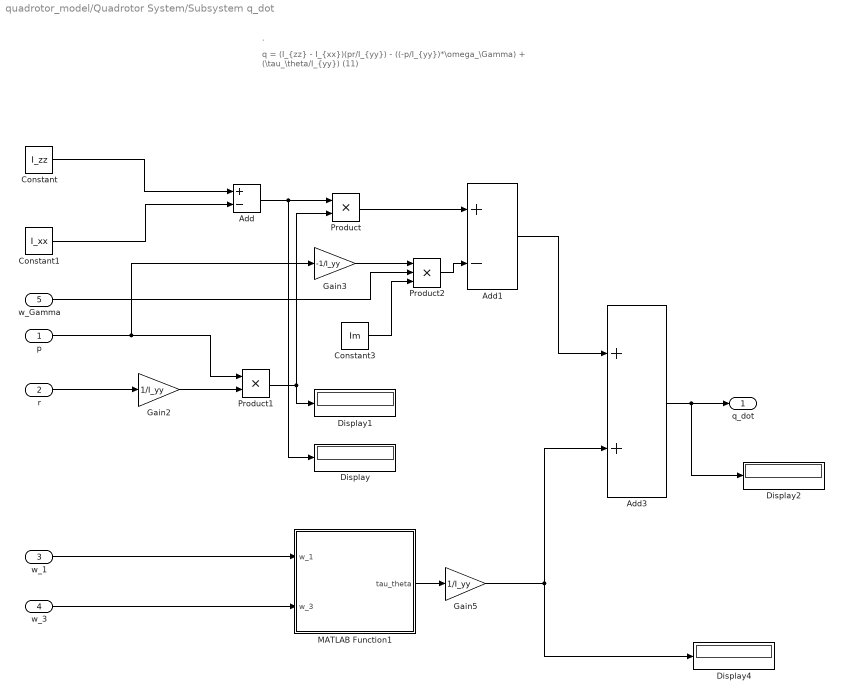
== system quadrotor_model/Quadrotor System/Subsystem q_dot ==
  note: q = (I_{zz} - I_{xx})(pr/I_{yy}) - ((-p/I_{yy})*\omega_\Gamma) + (\tau_\theta/I_{yy}) (11)
  note: .
  "p " : Inport
  r : Inport  Port=2
  w_1 : Inport  Port=3
  w_3 : Inport  Port=4
  "w_Gamma " : Inport  Port=5
  Add : Sum  Inputs=+-
  Add1 : Sum  Inputs=+-
  Add3 : Sum
  Constant : Constant  Value=I_zz
  Constant1 : Constant  Value=I_xx
  Constant3 : Constant  Value=Im
  Display{,1..2,4} (4 alike) : Display
  Gain2 : Gain  Gain=1/I_yy
  Gain3 : Gain  Gain=-1/I_yy
  Gain5 : Gain  Gain=1/I_yy
  MATLAB Function1 : MATLAB Function  TreatAsAtomicUnit=on
  Product : Product
  Product1 : Product
  Product2 : Product  Inputs=3
  q_dot : Outport
  wires:
  Constant/1 -> Add/1
  Constant1/1 -> Add/2
  Add/1 -> Display/1, Product/1
  Product1/1 -> Product/2, Display1/1
  Product/1 -> Add1/1
  Gain3/1 -> Product2/1
  Product2/1 -> Add1/2
  r/1 -> Gain2/1
  Gain2/1 -> Product1/2
  "p "/1 -> Gain3/1, Product1/1
  w_3/1 -> MATLAB Function1/2(w_3)
  MATLAB Function1/1(tau_theta) -> Gain5/1
  w_1/1 -> MATLAB Function1/1(w_1)
  Add1/1 -> Add3/1
  Add3/1 -> q_dot/1, Display2/1
  "w_Gamma "/1 -> Product2/2
  Gain5/1 -> Display4/1, Add3/2
  Constant3/1 -> Product2/3

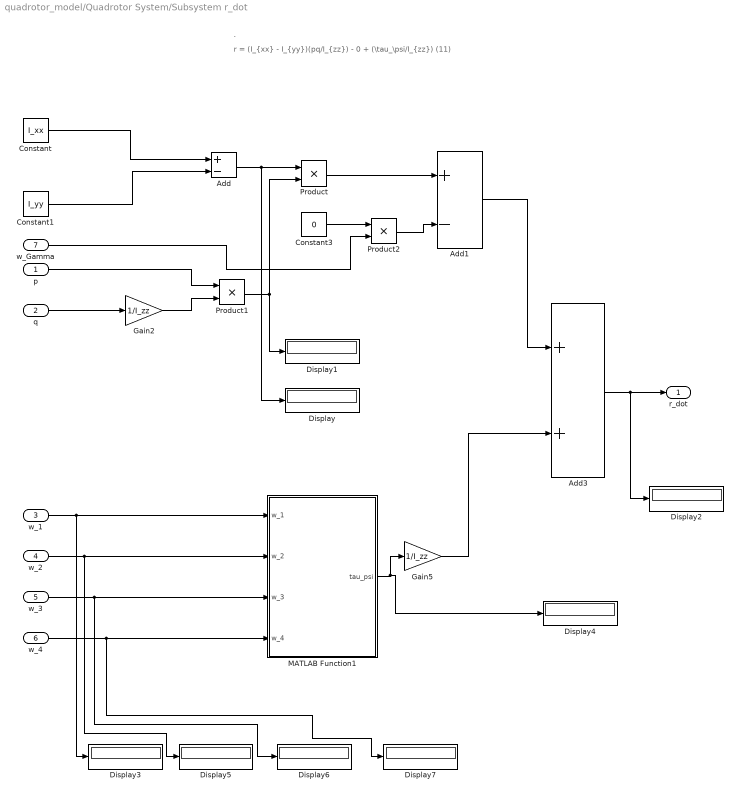
== system quadrotor_model/Quadrotor System/Subsystem r_dot ==
  note: r = (I_{xx} - I_{yy})(pq/I_{zz}) - 0 + (\tau_\psi/I_{zz}) (11)
  note: .
  "p " : Inport
  q : Inport  Port=2
  w_1 : Inport  Port=3
  w_2 : Inport  Port=4
  w_3 : Inport  Port=5
  w_4 : Inport  Port=6
  w_Gamma : Inport  Port=7
  Add : Sum  Inputs=+-
  Add1 : Sum  Inputs=+-
  Add3 : Sum
  Constant : Constant  Value=I_xx
  Constant1 : Constant  Value=I_yy
  Constant3 : Constant  Value=0
  Display{,1..7} (8 alike) : Display
  Gain2 : Gain  Gain=1/I_zz
  Gain5 : Gain  Gain=1/I_zz
  MATLAB Function1 : MATLAB Function  TreatAsAtomicUnit=on
  Product : Product
  Product1 : Product
  Product2 : Product
  r_dot : Outport
  wires:
  Constant/1 -> Add/1
  Constant1/1 -> Add/2
  Add/1 -> Display/1, Product/1
  Product1/1 -> Display1/1, Product/2
  Product/1 -> Add1/1
  Constant3/1 -> Product2/1
  Product2/1 -> Add1/2
  Add1/1 -> Add3/1
  Add3/1 -> Display2/1, r_dot/1
  "p "/1 -> Product1/1
  Gain2/1 -> Product1/2
  q/1 -> Gain2/1
  MATLAB Function1/1(tau_psi) -> Display4/1, Gain5/1
  w_1/1 -> MATLAB Function1/1(w_1), Display3/1
  w_2/1 -> MATLAB Function1/2(w_2), Display5/1
  w_4/1 -> MATLAB Function1/4(w_4), Display7/1
  w_Gamma/1 -> Product2/2
  Gain5/1 -> Add3/2
  w_3/1 -> MATLAB Function1/3(w_3), Display6/1

== system quadrotor_model/Quadrotor System/Subsystem theta ==
  note: \theta
  note: .
  note: \theta
  note: .
  note: \theta = q(C_\phi) - r(S_\theta) (4)
  q : Inport
  r : Inport  Port=2
  "phi " : Inport  Port=3
  Display1 : Display
  Display13 : Display
  Display14 : Display
  Integrator7 : Integrator  InitialConditionSource=external  InitialCondition=-0.09
  Pitch Initial : Constant  Value=pitch_i
  Product7 : Product
  Product8 : Product
  Z''4 : Sum  Inputs=-+
  sin 1 : Trigonometry  Operator=cos
  sin 2 : Trigonometry
  theta : Outport
  wires:
  "phi "/1 -> sin 1/1, sin 2/1
  r/1 -> Product7/2
  sin 1/1 -> Product8/1
  Product8/1 -> Display14/1, Z''4/2
  Z''4/1 -> Integrator7/1
  sin 2/1 -> Product7/1
  Product7/1 -> Display13/1, Z''4/1
  q/1 -> Product8/2
  Integrator7/1 -> Display1/1, theta/1
  Pitch Initial/1 -> Integrator7/2

== matlab function quadrotor_model/Quadrotor System/Subsystem r_dot/MATLAB Function1 ==
  data: w_1 input; w_2 input; w_3 input; tau_psi output; w_4 input
function tau_psi = fcn(w_1, w_2, w_3, w_4)
k = 2.980e-6; % Thrust factor of rotor (depends on density
              % geometry, etc) 
l = 0.225; % Linear distance from the centre of the rotor
           % to the centre of gravity    
b = 1.140e-7; % Drag constant
Im = 3.357e-5; % Inertia moment of the rotor
tau_psi = b*(-w_1^2 + w_2^2 - w_3^2 + w_4^2);
% tau_psi = (b * w_1^2 + Im) - (b * w_2^2 + Im) + (b * w_3^2 + Im) - (b * w_4^2 + Im);

== matlab function quadrotor_model/Quadrotor System/Subsystem p_dot/MATLAB Function ==
  data: w_2 input; w_4 input; tau_phi output
function tau_phi = fcn(w_2, w_4)
k = 2.980e-6; % Thrust factor of rotor (depends on density
              % geometry, etc) 
l = 0.225; % Linear distance from the centre of the rotor
           % to the centre of gravity          
tau_phi = l * k * (-w_2^2 + w_4^2);

== matlab function quadrotor_model/Quadrotor System/Subsystem q_dot/MATLAB Function1 ==
  data: w_1 input; w_3 input; tau_theta output
function tau_theta = fcn(w_1, w_3)
k = 2.980e-6; % Thrust factor of rotor (depends on density
              % geometry, etc) 
l = 0.225; % Linear distance from the centre of the rotor
           % to the centre of gravity          
tau_theta = l * k * (-w_1^2 + w_3^2);

== matlab function quadrotor_model/Quadrotor System/Thrust ==
  data: w_1 input; T output; w_2 input; w_3 input; w_4 input
function T = fcn(w_1, w_2, w_3, w_4)
k = 2.980e-6; % Thrust factor of rotor (depends on density
T = k * (w_1^2 + w_2^2 + w_3^2 + w_4^2);

== matlab function quadrotor_model/Quadrotor System/Gyroscope ==
  data: w_1 input; w_2 input; w_3 input; w_Gamma output; w_4 input
function w_Gamma = fcn(w_1, w_2, w_3, w_4)
    
w_Gamma = w_1 - w_2 + w_3 - w_4;
